simulink model "MapPIDLag"  (R2023a)
settings: Solver=VariableStepAuto  StartTime=0.0  StopTime=10.0  RelTol=1e-3
undefined symbols (not defined in the file or in its folder): DiscIntNeverNeededParam, MapPIDLag_H_den, MapPIDLag_H_num, MapPIDLag_Kaw, MapPIDLag_Kd, MapPIDLag_Ki, MapPIDLag_Kp, MapPIDLag_table, MapPIDLag_Tf, MapPIDLag_Ts_bp, MapPIDLag_Ts_ctrl, MapPIDLag_v_bp, Tdref_ay_bp_ms2, Tdref_table, Tdref_v_bp_ms
settings Model: Creator=Tan_Tram  LastModifiedBy=Tan_Tram

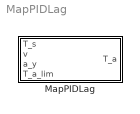
== system MapPIDLag ==
  MapPIDLag : Subsystem

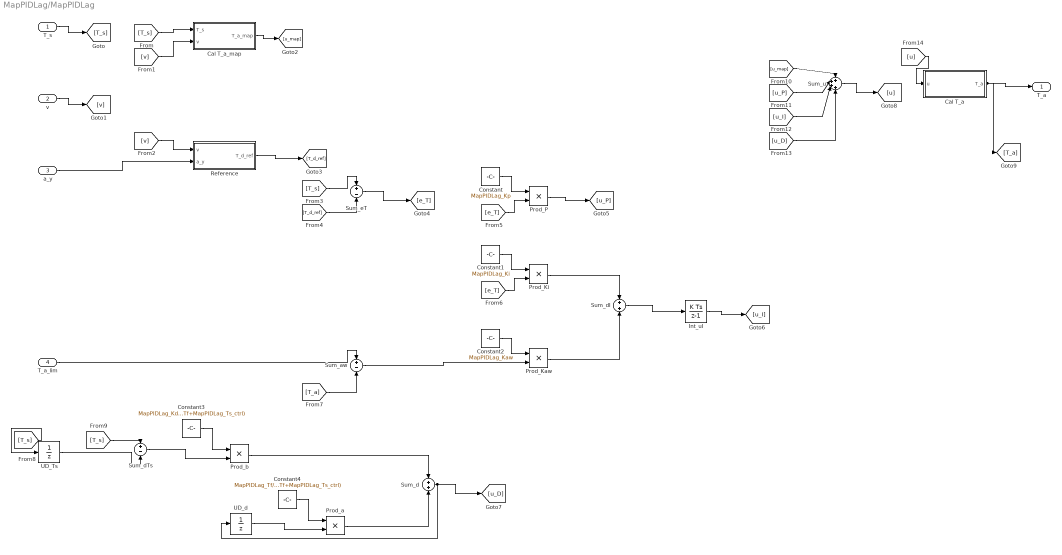
== system MapPIDLag/MapPIDLag ==
  T_s : Inport
  v : Inport  Port=2
  a_y : Inport  Port=3
  T_a_lim : Inport  Port=4
  Cal T_a : Subsystem
  Cal T_a_map : Subsystem
  Constant : Constant  Value=MapPIDLag_Kp
  Constant1 : Constant  Value=MapPIDLag_Ki
  Constant2 : Constant  Value=MapPIDLag_Kaw
  Constant3 : Constant  Value=MapPIDLag_Kd/(MapPIDLag_Tf+MapPIDLag_Ts_ctrl)
  Constant4 : Constant  Value=MapPIDLag_Tf/(MapPIDLag_Tf+MapPIDLag_Ts_ctrl)
  Int_uI : DiscreteIntegrator  gainval=1  SampleTime=MapPIDLag_Ts_ctrl  ICPrevOutput=DiscIntNeverNeededParam  ICPrevScaledInput=DiscIntNeverNeededParam
  Prod_Kaw : Product  Inputs=**
  Prod_Ki : Product  Inputs=**
  Prod_P : Product  Inputs=**
  Prod_a : Product  Inputs=**
  Prod_b : Product  Inputs=**
  Reference : Subsystem
  Sum_aw : Sum  Inputs=+-
  Sum_d : Sum
  Sum_dI : Sum
  Sum_dTs : Sum  Inputs=+-
  Sum_eT : Sum  Inputs=+-
  Sum_u : Sum  Inputs=++++
  UD_Ts : UnitDelay  SampleTime=MapPIDLag_Ts_ctrl  HasFrameUpgradeWarning=on
  UD_d : UnitDelay  SampleTime=MapPIDLag_Ts_ctrl  HasFrameUpgradeWarning=on
  T_a : Outport
  wires:
  T_s/1 -> [T_s]
  v/1 -> [v]
  [T_s] -> Cal T_a_map/1(T_s)
  [v] -> Cal T_a_map/2(v)
  Cal T_a_map/1(T_a_map) -> [u_map]
  [v] -> Reference/1(v)
  a_y/1 -> Reference/2(a_y)
  Reference/1(T_d_ref) -> [T_d_ref]
  [T_s] -> Sum_eT/1
  [T_d_ref] -> Sum_eT/2
  Sum_eT/1 -> [e_T]
  Constant/1 -> Prod_P/1
  [e_T] -> Prod_P/2
  Prod_P/1 -> [u_P]
  Constant1/1 -> Prod_Ki/1
  [e_T] -> Prod_Ki/2
  T_a_lim/1 -> Sum_aw/1
  [T_a] -> Sum_aw/2
  Constant2/1 -> Prod_Kaw/1
  Sum_aw/1 -> Prod_Kaw/2
  Prod_Ki/1 -> Sum_dI/1
  Prod_Kaw/1 -> Sum_dI/2
  Sum_dI/1 -> Int_uI/1
  Int_uI/1 -> [u_I]
  [T_s] -> UD_Ts/1
  [T_s] -> Sum_dTs/1
  UD_Ts/1 -> Sum_dTs/2
  Constant3/1 -> Prod_b/1
  Sum_dTs/1 -> Prod_b/2
  Constant4/1 -> Prod_a/1
  UD_d/1 -> Prod_a/2
  Prod_b/1 -> Sum_d/1
  Prod_a/1 -> Sum_d/2
  Sum_d/1 -> UD_d/1, [u_D]
  [u_map] -> Sum_u/1
  [u_P] -> Sum_u/2
  [u_I] -> Sum_u/3
  [u_D] -> Sum_u/4
  Sum_u/1 -> [u]
  [u] -> Cal T_a/1(u)
  Cal T_a/1(T_a) -> T_a/1, [T_a]

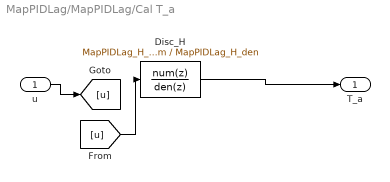
== system MapPIDLag/MapPIDLag/Cal T_a ==
  u : Inport
  Disc_H : DiscreteTransferFcn  Numerator=MapPIDLag_H_num  Denominator=MapPIDLag_H_den  SampleTime=MapPIDLag_Ts_ctrl
  T_a : Outport
  wires:
  u/1 -> [u]
  [u] -> Disc_H/1
  Disc_H/1 -> T_a/1

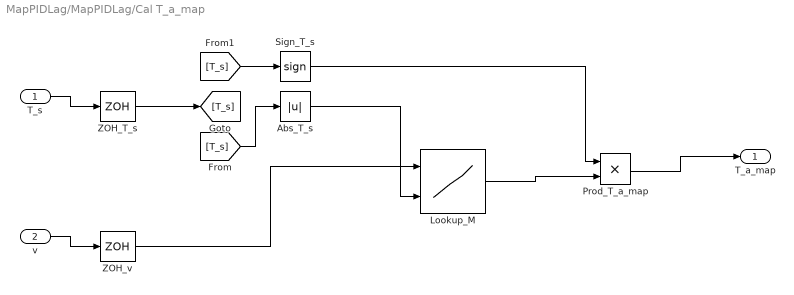
== system MapPIDLag/MapPIDLag/Cal T_a_map ==
  T_s : Inport
  v : Inport  Port=2
  Abs_T_s : Abs  SaturateOnIntegerOverflow=off
  Lookup_M : Lookup_n-D  BreakpointsForDimension1=MapPIDLag_v_bp  BreakpointsForDimension2=MapPIDLag_Ts_bp  BreakpointsForDimension3=[5, 7]  Table=MapPIDLag_table  ExtrapMethod=Clip  InternalRulePriority=Speed  RndMeth=Simplest
      settings: InputPortMap=u0,u1
  Prod_T_a_map : Product  Inputs=**
  Sign_T_s : Signum
  ZOH_T_s : ZeroOrderHold  SampleTime=MapPIDLag_Ts_ctrl
  ZOH_v : ZeroOrderHold  SampleTime=MapPIDLag_Ts_ctrl
  T_a_map : Outport
  wires:
  T_s/1 -> ZOH_T_s/1
  v/1 -> ZOH_v/1
  ZOH_T_s/1 -> [T_s]
  [T_s] -> Abs_T_s/1
  [T_s] -> Sign_T_s/1
  ZOH_v/1 -> Lookup_M/1
  Abs_T_s/1 -> Lookup_M/2
  Sign_T_s/1 -> Prod_T_a_map/1
  Lookup_M/1 -> Prod_T_a_map/2
  Prod_T_a_map/1 -> T_a_map/1

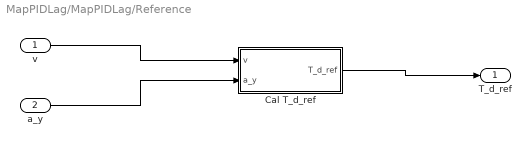
== system MapPIDLag/MapPIDLag/Reference ==
  v : Inport
  a_y : Inport  Port=2
  Cal T_d_ref : Subsystem
  T_d_ref : Outport
  wires:
  Cal T_d_ref/1(T_d_ref) -> T_d_ref/1
  a_y/1 -> Cal T_d_ref/2(a_y)
  v/1 -> Cal T_d_ref/1(v)

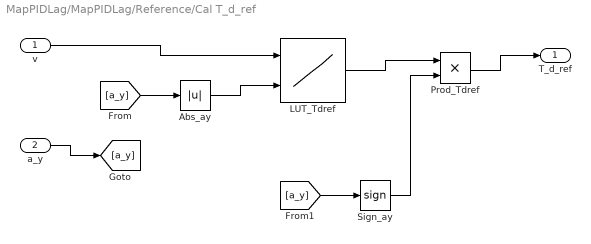
== system MapPIDLag/MapPIDLag/Reference/Cal T_d_ref ==
  v : Inport
  a_y : Inport  Port=2
  Abs_ay : Abs  SaturateOnIntegerOverflow=off
  LUT_Tdref : Lookup_n-D  BreakpointsForDimension1=Tdref_v_bp_ms  BreakpointsForDimension2=Tdref_ay_bp_ms2  Table=Tdref_table  ExtrapMethod=Clip  InternalRulePriority=Speed  RndMeth=Simplest
      settings: InputPortMap=u0,u1
  Prod_Tdref : Product  Inputs=**
  Sign_ay : Signum
  T_d_ref : Outport
  wires:
  Prod_Tdref/1 -> T_d_ref/1
  Sign_ay/1 -> Prod_Tdref/2
  LUT_Tdref/1 -> Prod_Tdref/1
  [a_y] -> Sign_ay/1
  Abs_ay/1 -> LUT_Tdref/2
  [a_y] -> Abs_ay/1
  v/1 -> LUT_Tdref/1
  a_y/1 -> [a_y]
